simulink model "dynamic_text"  (Simulink 8.1)
settings: Solver=ode4  SolverMode=SingleTasking  StartTime=0.0  StopTime=inf  FixedStep=0.0005  RelTol=1e-3
model workspace (MAT data in the model file):
  BKIN_STEP_TIME = 0.0005
  col_x = 1
  col_y = 2
  ROTATION = 3
  WIDTH = 4
  HEIGHT = 5
  LABEL_TEXT = 7
  LABEL_COLOR = 8
  LABEL_HEIGHT = 9
  TARG_COLOR : num (value not decoded)
StartFcn:
  |  warndlg('Dexterit-E models cannot run under simulation. Please compile your model and run it from within Dexterit-E.');set_param(bdroot,'SimulationCommand','stop')
libraries: General x3, Video x2, KINARM_general x1, xpclib x1
CloseFcn:
  | rtwprivate ssgencode ModelCloseRequest b2lab2d
settings Model: Creator=Chris Grebeldinger  LastModifiedBy=User  ModifiedComment=chris -- Wed Feb 16 09:18:30 2005 -- Version 1.1384  ModifiedHistory=Feb 16/05 - Add error repeat, add offset ramp  ExtModeArmWhenConnect=off  ExtModeLogAll=off  BufferReuse=off
settings DataIOCC: LimitDataPoints=off  SaveOutput=off  SaveTime=off  SignalLoggingName=sigsOut
settings OptimizationCC: BlockReduction=off  BooleanDataType=off  OptimizeBlockIOStorage=off  BufferReuse=off  ExpressionFolding=off  FoldNonRolledExpr=off  LocalBlockOutputs=off  InitFltsAndDblsToZero=on
settings DebuggingCC: SaveWithParameterizedLinksMsg=none  SignalResolutionControl=TryResolveAllWithWarning  SolverPrmCheckMsg=none  MultiTaskDSMMsg=warning  MultiTaskCondExecSysMsg=none  StrictBusMsg=None
settings HardwareCC: ProdIntDivRoundTo=Zero  ProdEndianess=LittleEndian  ProdHWDeviceType=Generic->32-bit x86 compatible  TargetHWDeviceType=32-bit Generic
settings SFSimCC: SimParseCustomCode=off
settings RTWCC: SystemTargetFile=xpctarget.tlc  TemplateMakefile=xpc_default_tmf  Description=xPC Target  ProcessScript=xpctarget_make_rtw_hook  IncludeERTFirstTime=on  RTWCompilerOptimization=On
settings CodeAppCC: MaxIdLength=63
settings xpcTargetCC: TargetFcnLib=ansi_tfl_tmw.mat  CodeReplacementLibrary=XPC_BLAS  ParMdlRefBuildCompliant=on  ConcurrentExecutionCompliant=on  CombineSignalStateStructs=off  MATLABClassNameForMDSCustomization=xpcAperiodicCustomization  GRTInterface=on  GenerateAllocFcn=off  xPCTaskExecutionProfile=off  xPCRL32EventNumber=5000  xPCisDownloadable=off  xPCLoadParamSetFile=off  xPCConcurrentTasks=off  xPCEnableSFAnimation=off

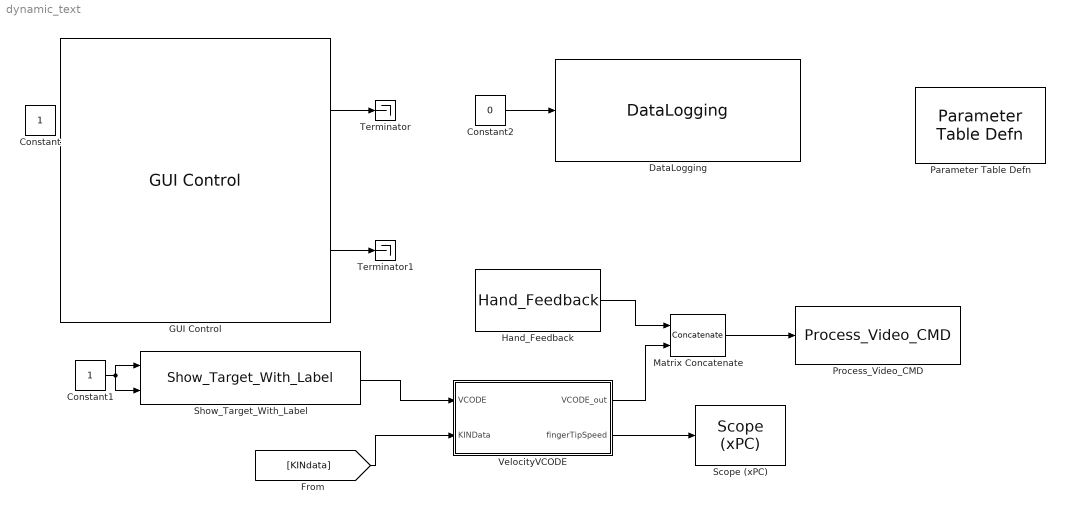
== system dynamic_text ==
  Constant1 : Constant
  Constant2 : Constant  Value=0
  DataLogging : General/DataLogging  log_event_codes=off  log_analog_inputs=off
      link override Poll KINARM/ZeroEPTorque: Value=[0 0 0 0]
      link override Poll KINARM/ZeroTorque: Value=[0 0 0 0]
  GUI Control : General/GUI Control  target_type_str=Circle  Target_Type=1  XYcols=[1 2]  Vcols=3  Lcols=4  indices_padding=[0 0 0 0;0 0 0 0]  task_version=1.0  show_repeat_trial_flag=off
  Hand_Feedback : KINARM_general/Hand_Feedback  feedback_cntl_src=none
  Matrix Concatenate : Concatenate  Mode=Multidimensional array
  Parameter Table Defn : General/Parameter Table Defn  ShowInLibBrowser=0
  Process_Video_CMD : Video/Process_Video_CMD
  "Scope (xPC) " : xpclib/Misc./Scope (xPC)   scopeno=1  scopetype=Target  autostart=on  viewmode=Numerical  formatstr='%15.6f'  grid=on  ylimits=[0,0]  nosamples=250  noprepostsamples=0  interleave=1  triggermode=FreeRun  triggersignal=1  trigsignalfromport=off  triggerlevel=0.0  triggerslope=Either  triggerscope=1  triggersample=0  filename=data.dat  mode=Lazy  writesize=512  autorestart=off  dynamicfilemode=off  maxwritefilesize=512*1024^2
  Show_Target_With_Label : Video/Show_Target_With_Label  target_type=Rectangle  num_states=1  attribcol1=[TARG_COLOR 0 0 WIDTH HEIGHT ROTATION LABEL_TEXT LABEL_COLOR LABEL_HEIGHT]  attribcol2=[6 6 0 3 0 0 0 0 0]  attribcol3=[0 0 0 0 0 0 0 0 0]  attribcol4=[0 0 0 0 0 0 0 0 0]  attribcol5=[0 0 24 0 0 0 0 0 0]  stateindices_padding=[0 0;0 0;0 0;0 0;0 0]  source=dialog  opacity=100  target_display=Both subject and operator displays
  Terminator : Terminator
  Terminator1 : Terminator
  VelocityVCODE : MATLAB Function  TreatAsAtomicUnit=on
  Constant : Constant  IOType=siggen
  wires:
  Hand_Feedback/1 -> Matrix Concatenate/1
  VelocityVCODE/1(VCODE_out) -> Matrix Concatenate/2
  Matrix Concatenate/1 -> Process_Video_CMD/1
  [KINdata] -> VelocityVCODE/2(KINData)
  VelocityVCODE/2(fingerTipSpeed) -> "Scope (xPC) "/1
  Constant1/1 -> Show_Target_With_Label/1, Show_Target_With_Label/2
  Show_Target_With_Label/1 -> VelocityVCODE/1(VCODE)
  Constant2/1 -> DataLogging/1
  GUI Control/1 -> Terminator/1
  GUI Control/2 -> Terminator1/1

== matlab function VelocityVCODE ==
  settings: fimath=|
      | fimath(...
      | 'RoundMode', 'floor',...
      | 'OverflowMode', 'wrap',...
      | 'ProductMode', 'KeepLSB', 'ProductWordLength', 32,...
      | 'SumMode', 'KeepLSB', 'SumWordLength', 32,...
      | 'CastBeforeSum', false)
  data: VCODE input double; VCODE_out output double; KINData input double; fingerTipSpeed output double
function [VCODE_out, fingerTipSpeed]= velocityVCode(VCODE, KINData)

arm = KINData(3,1);

handVelX = KINData(arm,25);
handVelY = KINData(arm,26);

fingerTipSpeed = (sqrt(handVelX^2 + handVelY^2)) * 100;

%don't show a zero, show a blank in the 100's position
if fingerTipSpeed < 100
	VCODE(15) = 32; %' ' space
else
	VCODE(15) = getChar(fingerTipSpeed, 100);
end

%don't show a zero, show a blank in the 10's position
if fingerTipSpeed < 10
	VCODE(16) = 32; %' ' space
else
	VCODE(16) = getChar(fingerTipSpeed, 10);
end

VCODE(17) = getChar(fingerTipSpeed, 1);
VCODE(18) = 32;  %' ' space
VCODE(19) = 99;  % c
VCODE(20) = 109; % m
VCODE(21) = 47;  % \
VCODE(22) = 115; % s
VCODE(23) = 0;	 %terminate the new string

VCODE_out=VCODE;
end

function cc = getChar(number, dec)
	%in simulink there is no nice way to convert a number to s string
	%so what we are doing here is converting a single digit to a character.
	%48 is ascii for '0', so this gets the least significant digit before 
	%the decimal and converts to ascii.
    cc = floor(mod(number / dec, 10)) + 48;
end
